simulink model "tema2"  (R2024b)
settings: Solver=VariableStepAuto  StartTime=0.0  StopTime=10.0  RelTol=1e-3
settings Model: Creator=alex_  LastModifiedBy=alex_

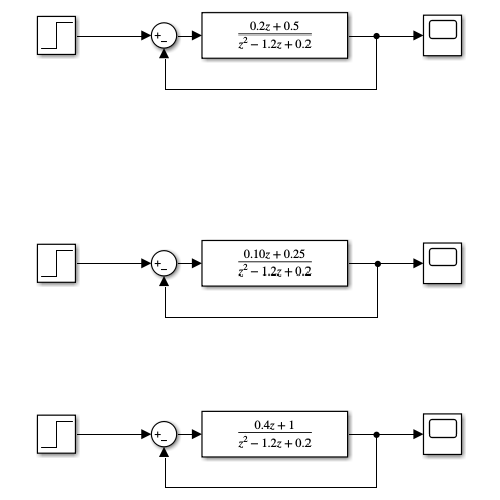
[thumbnail: Simulink's stored preview of the top-level diagram]
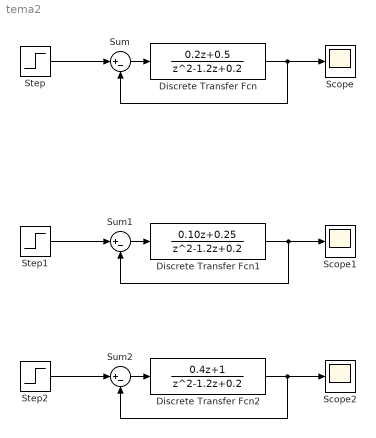
== system tema2 ==
  Discrete Transfer Fcn : DiscreteTransferFcn  Numerator=[0.2 0.5]  Denominator=[1 -1.2 0.2]
  Discrete Transfer Fcn1 : DiscreteTransferFcn  Numerator=[0.10 0.25]  Denominator=[1 -1.2 0.2]
  Discrete Transfer Fcn2 : DiscreteTransferFcn  Numerator=[0.4 1]  Denominator=[1 -1.2 0.2]
  Scope : Scope
  Scope1 : Scope
  Scope2 : Scope
  Step : Step  Time=0  SampleTime=0
  Step1 : Step  Time=0  SampleTime=0
  Step2 : Step  Time=0  SampleTime=0
  Sum : Sum  Inputs=|+-
  Sum1 : Sum  Inputs=|+-
  Sum2 : Sum  Inputs=|+-
  wires:
  Step/1 -> Sum/1
  Sum/1 -> Discrete Transfer Fcn/1
  Step1/1 -> Sum1/1
  Sum1/1 -> Discrete Transfer Fcn1/1
  Step2/1 -> Sum2/1
  Sum2/1 -> Discrete Transfer Fcn2/1
  Discrete Transfer Fcn2/1 -> Sum2/2, Scope2/1
  Discrete Transfer Fcn1/1 -> Sum1/2, Scope1/1
  Discrete Transfer Fcn/1 -> Sum/2, Scope/1
